simulink model "ace_id_arduino"  (R2026a)
settings: Solver=FixedStepDiscrete  StopTime=C.id_T  FixedStep=0.02  EnableMultiTasking=on
PreLoadFcn:
  | ace_params;
InitFcn:
  | ace_params;
values from neighbouring files (symbols this model uses):
  C = struct()    [ace_params.m]    (also in build_ace_sysid_pipeline.m = evalin('base', 'C'))
libraries: arduinolib x3, arduinosensorlib x1
settings Model: SimulationMode=external  SILPILModeSetting=veronly  ExtModeTrigDuration=2  Creator=00782620  LastModifiedBy=00782620
settings HardwareCC: ProdBitPerInt=16.0  ProdBitPerPointer=16.0  ProdBitPerSizeT=16.0  ProdBitPerPtrDiffT=16.0  ProdWordSize=8.0  ProdHWDeviceType=Atmel->AVR
settings RTWCC: SystemTargetFile=ert.tlc  HardwareBoard=Arduino Uno  TLCOptions=-aInlineSetEventsForThisBaseRateFcn=TLC_FALSE -aSuppressMultiTaskScheduler=TLC_FALSE -aRateBasedStepFcn=1  Toolchain=Arduino AVR  BuildConfiguration=Faster Runs  Description=Embedded Coder
settings ERTTargetCC: ExtModeTransport=3.0  ExtModeAutomaticAllocSize=off  ExtModeStaticAllocSize=250.0  SupportContinuousTime=on  SupportVariableSizeSignals=on

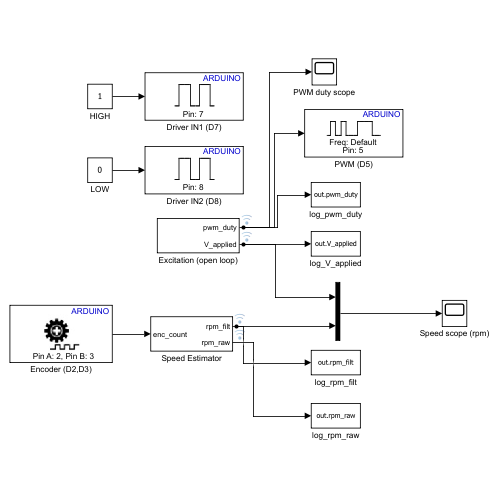
[thumbnail: Simulink's stored preview of the top-level diagram]
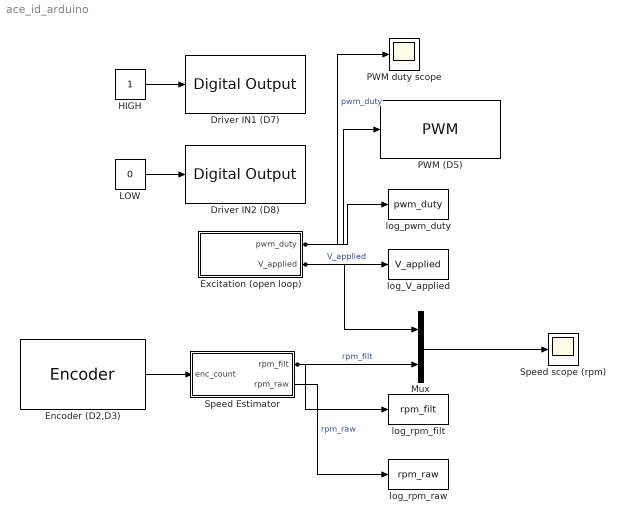
== system ace_id_arduino ==
  Driver IN1 (D7) : arduinolib/Digital Output  pinNumber=7  Direction=output  blockPlatform=arduino
  Driver IN2 (D8) : arduinolib/Digital Output  pinNumber=8  Direction=output  blockPlatform=arduino
  Encoder (D2,D3) : arduinosensorlib/Encoder  InputA=2  InputB=3  Mode=No reset  SampleTime=0.02
  Excitation (open loop) : Subsystem
  HIGH : Constant  SampleTime=C.Ts
  LOW : Constant  Value=0  SampleTime=C.Ts
  Mux : Mux  Inputs=2
  PWM (D5) : arduinolib/PWM  pinNumber=5  frequencyType=Default  desiredFrequency=490.2  achievableFrequency=490.2
  PWM duty scope : Scope
  Speed Estimator : Subsystem
  Speed scope (rpm) : Scope
  log_V_applied : ToWorkspace  VariableName=V_applied  SaveFormat=Timeseries  SampleTime=-1
  log_pwm_duty : ToWorkspace  VariableName=pwm_duty  SaveFormat=Timeseries  SampleTime=-1
  log_rpm_filt : ToWorkspace  VariableName=rpm_filt  SaveFormat=Timeseries  SampleTime=-1
  log_rpm_raw : ToWorkspace  VariableName=rpm_raw  SaveFormat=Timeseries  SampleTime=-1
  wires:
  Mux/1 -> Speed scope (rpm)/1
  Encoder (D2,D3)/1 -> Speed Estimator/1(enc_count)
  HIGH/1 -> Driver IN1 (D7)/1
  LOW/1 -> Driver IN2 (D8)/1
  Excitation (open loop)/1(pwm_duty) -> PWM (D5)/1, log_pwm_duty/1, PWM duty scope/1  "pwm_duty"
  Excitation (open loop)/2(V_applied) -> log_V_applied/1, Mux/1  "V_applied"
  Speed Estimator/1(rpm_filt) -> log_rpm_filt/1, Mux/2  "rpm_filt"
  Speed Estimator/2(rpm_raw) -> log_rpm_raw/1  "rpm_raw"

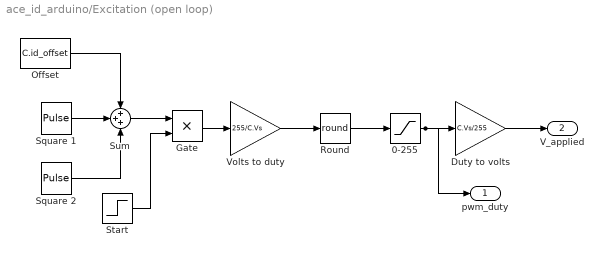
== system ace_id_arduino/Excitation (open loop) ==
  0-255 : Saturate  UpperLimit=255  LowerLimit=0
  Duty to volts : Gain  Gain=C.Vs/255
  Gate : Product
  Offset : Constant  Value=C.id_offset  SampleTime=C.Ts
  Round : Rounding  Operator=round
  Square 1 : DiscretePulseGenerator  Amplitude=C.id_amp1  Period=C.id_per1  PulseWidth=C.id_per1/2  SampleTime=C.Ts
  Square 2 : DiscretePulseGenerator  Amplitude=C.id_amp2  Period=C.id_per2  PulseWidth=C.id_per2/2  SampleTime=C.Ts
  Start : Step  Time=C.id_start  SampleTime=C.Ts
  Sum : Sum  Inputs=+++
  Volts to duty : Gain  Gain=255/C.Vs
  pwm_duty : Outport
  V_applied : Outport  Port=2
  wires:
  Offset/1 -> Sum/1
  Round/1 -> 0-255/1
  Sum/1 -> Gate/1
  Volts to duty/1 -> Round/1
  0-255/1 -> pwm_duty/1, Duty to volts/1
  Square 2/1 -> Sum/3
  Square 1/1 -> Sum/2
  Gate/1 -> Volts to duty/1
  Start/1 -> Gate/2
  Duty to volts/1 -> V_applied/1

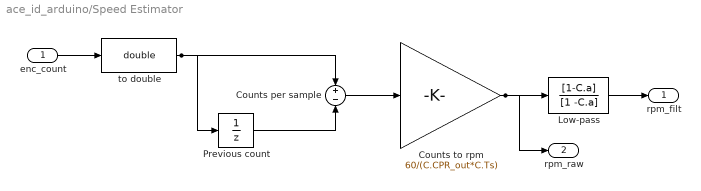
== system ace_id_arduino/Speed Estimator ==
  enc_count : Inport
  Counts per sample : Sum  Inputs=+-
  Counts to rpm : Gain  Gain=60/(C.CPR_out*C.Ts)
  Low-pass : DiscreteTransferFcn  Numerator=[1-C.a]  Denominator=[1 -C.a]  SampleTime=C.Ts
  Previous count : UnitDelay  SampleTime=C.Ts
  to double : DataTypeConversion  OutDataTypeStr=double  SaturateOnIntegerOverflow=off  RndMeth=Floor
  rpm_filt : Outport
  rpm_raw : Outport  Port=2
  wires:
  Counts to rpm/1 -> rpm_raw/1, Low-pass/1
  Counts per sample/1 -> Counts to rpm/1
  Previous count/1 -> Counts per sample/2
  enc_count/1 -> to double/1
  to double/1 -> Previous count/1, Counts per sample/1
  Low-pass/1 -> rpm_filt/1
